simulink model "DAB_SPS_OL"  (R2024a)
settings: Solver=VariableStepAuto  StartTime=0.0  StopTime=1  RelTol=1e-3
libraries: spsIGBTDiodeLib x4, spsMosfetLib x4, spsSeriesRLCBranchLib x4, spsCurrentMeasurementLib x1, spsDCVoltageSourceLib x1, spsMeanLib x1, spsVariableRatioTransformerLib x1, spsVoltageMeasurementLib x1, sps_lib x1
settings Model: Creator=hp  LastModifiedBy=DIPAK PRODHANI

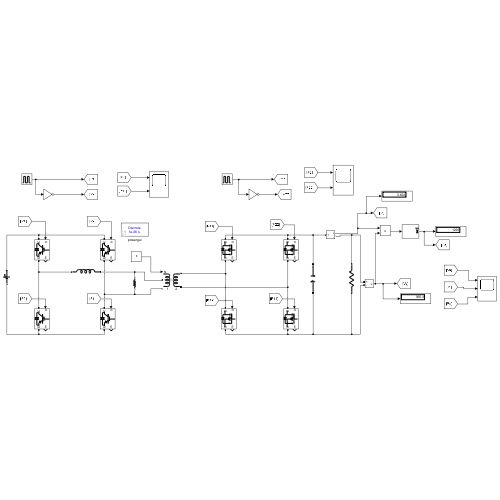
[thumbnail: Simulink's stored preview of the top-level diagram]
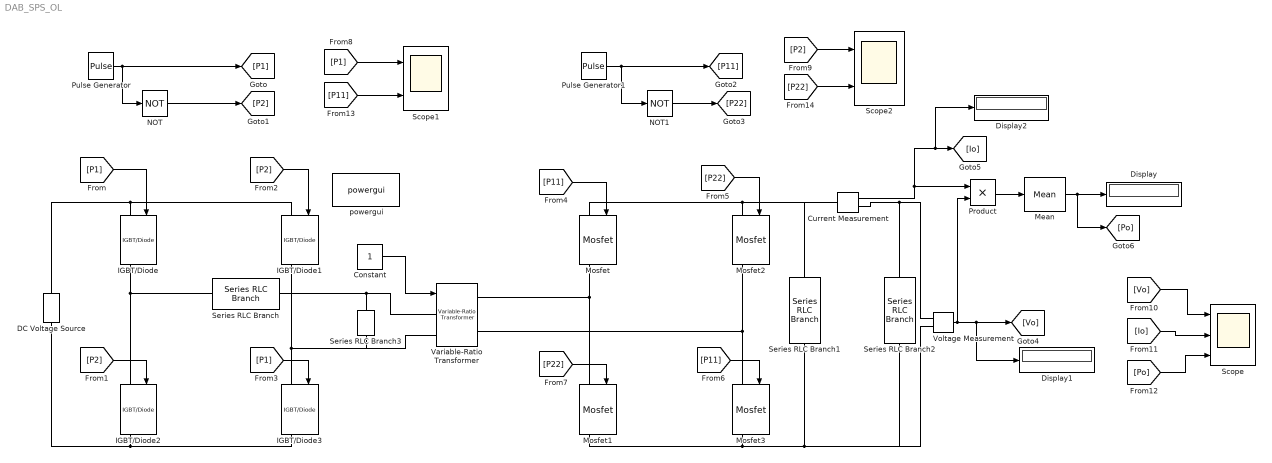
== system DAB_SPS_OL ==
  Constant : Constant
  Current Measurement : spsCurrentMeasurementLib/Current Measurement  PhasorSimulation=off  OutputType=Complex  PSBequivalent=0
  DC Voltage Source : spsDCVoltageSourceLib/DC Voltage Source  Amplitude=400  Measurements=None
  Display : Display
  Display1 : Display
  Display2 : Display
  IGBT/Diode{,1..3} (4 alike) : spsIGBTDiodeLib/IGBT//Diode  Ron=1e-3  Rs=1e5  Cs=inf  Measurements=on
  Mean : spsMeanLib/Mean  Freq=50  Vinit=0  Ts=0
  Mosfet{,1..3} (4 alike) : spsMosfetLib/Mosfet  Ron=0.1  Lon=0  Rd=0.01  Vfd=0  IC=0  Rs=1e5  Cs=inf  Measurements=on
  NOT : Logic  Operator=NOT  IconShape=distinctive  AllPortsSameDT=off  OutDataTypeStr=boolean
  NOT1 : Logic  Operator=NOT  IconShape=distinctive  AllPortsSameDT=off  OutDataTypeStr=boolean
  Product : Product
  Pulse Generator : DiscretePulseGenerator  PulseType=Time based  Period=1/20000  PulseWidth=50
  Pulse Generator1 : DiscretePulseGenerator  PulseType=Time based  Period=1/20000  PulseWidth=50  PhaseDelay=1.39e-6
  Scope : Scope  NumInputPorts=3
  Scope1 : Scope  NumInputPorts=2
  Scope2 : Scope  NumInputPorts=2
  Series RLC Branch : spsSeriesRLCBranchLib/Series RLC Branch  LConnTagsString=__new0  RConnTagsString=__new0  BranchType=L  Resistance=0.01  Inductance=100e-6  SetiL0=off  InitialCurrent=0  Capacitance=1e-6  Setx0=off  InitialVoltage=0  Measurements=None
  Series RLC Branch1 : spsSeriesRLCBranchLib/Series RLC Branch  LConnTagsString=__new0  RConnTagsString=__new0  BranchType=C  Resistance=1  Inductance=1e-3  SetiL0=off  InitialCurrent=0  Capacitance=1000e-6  Setx0=off  InitialVoltage=0  Measurements=None
  Series RLC Branch2 : spsSeriesRLCBranchLib/Series RLC Branch  LConnTagsString=__new0  RConnTagsString=__new0  BranchType=R  Resistance=100  Inductance=1e-3  SetiL0=off  InitialCurrent=0  Capacitance=1e-6  Setx0=off  InitialVoltage=0  Measurements=None
  Series RLC Branch3 : spsSeriesRLCBranchLib/Series RLC Branch  LConnTagsString=__new0  RConnTagsString=__new0  BranchType=R  Resistance=100  Inductance=100e-6  SetiL0=off  InitialCurrent=0  Capacitance=1e-6  Setx0=off  InitialVoltage=0  Measurements=None
  Variable-Ratio Transformer : spsVariableRatioTransformerLib/Variable-Ratio Transformer
      settings: LibrarySourceBlock=|
      | sps_lib/Passives/Variable-Ratio
      | Transformer
  Voltage Measurement : spsVoltageMeasurementLib/Voltage Measurement  PhasorSimulation=off  OutputType=Complex  PSBequivalent=0
  powergui : sps_lib/powergui  Priority=1  SimulationMode=Discrete  SampleTime=1e-6  frequency=60  Iterations=50  frequencyindice=0  Pbase=100e6  ErrMax=1e-4  UnitsV=kV  UnitsW=MW  buscounter=0  FunctionMessages=off  echomessages=off  EnableUseOfTLC=off  CurrentSourceSwitches=off  DisableSnubberDevices=off  DisableRonSwitches=off  DisableVfSwitches=off  DisplayEquations=off  AutomaticDiscreteSolvers=off  SolverType=Tustin/Backward Euler (TBE)  Interpol=off  ExternalGateDelay=off  methode=off  Ts=100  x0status=blocks  SPID=on  SwTol=0  HookPort=off  NonlinearTolerance=1e-4  nMaxIteration=100  ContinueOnMaxIteration=off  RestoreLinks=warning  ResistiveCurrentMeasurement=off  Frange=[0:2:500]  Ylog=off  Xlog=on  ShowGrid=off  save=off  variable=ZData  structure=0  ZoomFFT=off  StartTime=0.0  cycles=1  DisplayStyle=1  fundamental=60  FreqAxis=off  MaxFrequency=1000  frequencyindicesteady=1  RmsSteady=1  display=off
  wires:
  NOT/1 -> [P2]
  [P1] -> IGBT/Diode3/1
  [P2] -> IGBT/Diode1/1
  [P1] -> IGBT/Diode/1
  [P2] -> IGBT/Diode2/1
  Voltage Measurement/1 -> Product/2, [Vo], Display1/1
  Pulse Generator/1 -> [P1], NOT/1
  Constant/1 -> Variable-Ratio Transformer/1
  Current Measurement/1 -> Display2/1, [Io], Product/1
  Product/1 -> Mean/1
  Mean/1 -> [Po], Display/1
  Pulse Generator1/1 -> [P11], NOT1/1
  NOT1/1 -> [P22]
  [P22] -> Mosfet1/1
  [P11] -> Mosfet3/1
  [P22] -> Mosfet2/1
  [P11] -> Mosfet/1
  [P1] -> Scope1/1
  [Io] -> Scope/2
  [Vo] -> Scope/1
  [Po] -> Scope/3
  [P22] -> Scope2/2
  [P11] -> Scope1/2
  [P2] -> Scope2/1
  connections:
  IGBT/Diode2/LConn1 -- Series RLC Branch/LConn1 -- IGBT/Diode/RConn1
  IGBT/Diode3/LConn1 -- Variable-Ratio Transformer/LConn2 -- Series RLC Branch3/RConn1 -- IGBT/Diode1/RConn1
  IGBT/Diode/LConn1 -- DC Voltage Source/RConn1 -- IGBT/Diode1/LConn1
  IGBT/Diode2/RConn1 -- DC Voltage Source/LConn1 -- IGBT/Diode3/RConn1
  Series RLC Branch/RConn1 -- Variable-Ratio Transformer/LConn1 -- Series RLC Branch3/LConn1
  Mosfet1/LConn1 -- Mosfet/RConn1 -- Variable-Ratio Transformer/RConn1
  Mosfet3/LConn1 -- Variable-Ratio Transformer/RConn2 -- Mosfet2/RConn1
  Mosfet/LConn1 -- Current Measurement/LConn1 -- Series RLC Branch1/LConn1 -- Mosfet2/LConn1
  Mosfet1/RConn1 -- Series RLC Branch2/RConn1 -- Voltage Measurement/LConn2 -- Series RLC Branch1/RConn1 -- Mosfet3/RConn1
  Series RLC Branch2/LConn1 -- Current Measurement/RConn1 -- Voltage Measurement/LConn1
